simulink model "buck_closedloop_test"  (R2026a)
settings: Solver=VariableStepAuto  StopTime=0.005
libraries: cstblocks_lti x2
settings Model: Creator=raffaellamoccia  LastModifiedBy=raffaellamoccia

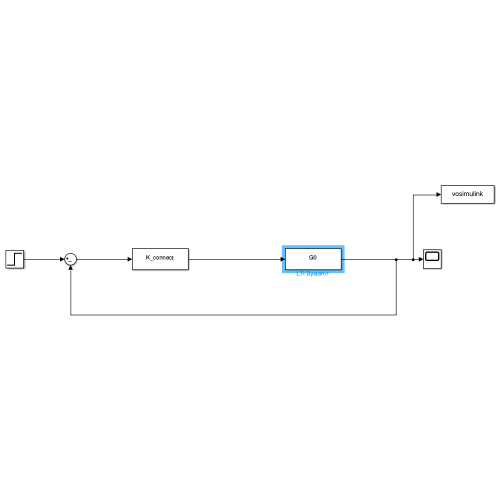
[thumbnail: Simulink's stored preview of the top-level diagram]
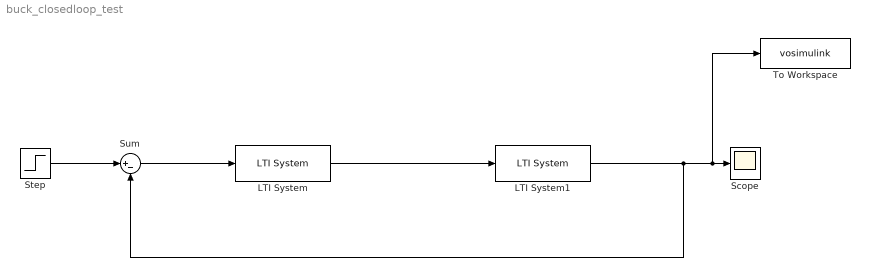
== system buck_closedloop_test ==
  LTI System : cstblocks_lti/LTI System  sys=K_connect  IC=[]  PadeOrder=0
      settings: LibrarySourceBlock=cstblocks/LTI System
  LTI System1 : cstblocks_lti/LTI System  sys=G0  IC=[]  PadeOrder=0
      settings: LibrarySourceBlock=cstblocks/LTI System
  Scope : Scope
      settings: ActiveDisplayYMinimum=4.9350867340038054  ActiveDisplayYMaximum=5.1136387408520605
  Step : Step  Time=0  FinalValue=5  SampleTime=0
  Sum : Sum  Inputs=|+-
  To Workspace : ToWorkspace  VariableName=vosimulink  SaveFormat=Timeseries  SampleTime=-1
  wires:
  Step/1 -> Sum/1
  Sum/1 -> LTI System/1
  LTI System/1 -> LTI System1/1
  LTI System1/1 -> Sum/2, To Workspace/1, Scope/1
